simulink model "tcptank"  (R2024a)
settings: Solver=ode45  StartTime=0.0  StopTime=200.0  RelTol=1e-3  EnableMultiTasking=on
undefined symbols (not defined in the file): DiscIntNeverNeededParam, Ts
libraries: instrumentlib x4, simulink x3, rllib x1
settings Model: Creator=The MathWorks, Inc.  LastModifiedBy=Administrator
settings SolverCC: AlgebraicLoopSolver=TrustRegion
settings DataIOCC: LimitDataPoints=on  SaveFormat=Array  ReturnWorkspaceOutputs=off  SignalLoggingName=logsOut
settings OptimizationCC: ExpressionDepthLimit=2147483647  InitFltsAndDblsToZero=on  LifeSpan=inf
settings DebuggingCC: SaveWithParameterizedLinksMsg=none  UnderspecifiedInitializationDetection=Classic  MergeDetectMultiDrivingBlocksExec=none  SignalResolutionControl=TryResolveAllWithWarning  MultiTaskDSMMsg=warning  FcnCallInpInsideContextMsg=warning  UnconnectedInputMsg=warning  UnconnectedOutputMsg=warning  UnconnectedLineMsg=warning  AllowSymbolicDim=off  StateNameClashWarn=warning  SFUnexpectedBacktrackingDiag=warning  SFNoUnconditionalDefaultTransitionDiag=warning  SFExecutionAtInitializationDiag=none  ArithmeticOperatorsInVariantConditions=warning
settings HardwareCC: ProdBitPerPointer=32  ProdBitPerSizeT=32  ProdBitPerPtrDiffT=32  ProdLargestAtomicFloat=None  ProdIntDivRoundTo=Undefined  ProdEndianess=Unspecified  ProdWordSize=32  ProdHWDeviceType=Specified
settings ModelReferenceCC: EnableRefExpFcnMdlSchedulingChecks=on  PropagateSignalLabelsOutOfModel=off
settings SFSimCC: SimUseLocalCustomCode=off
settings RTWCC: RTWUseLocalCustomCode=off  GPUComputeCapability=3.5
settings CodeAppCC: StateflowObjectComments=on
settings GRTTargetCC: TargetFcnLib=ansi_tfl_tmw.mat  TargetLangStandard=C89/C90 (ANSI)  CombineOutputUpdateFcns=off  GRTInterface=on
settings ConfigComp: CovMetricSettings=dw  CovSaveCumulativeToWorkspaceVar=on  CovSaveSingleToWorkspaceVar=on  CovExternalEMLEnable=off

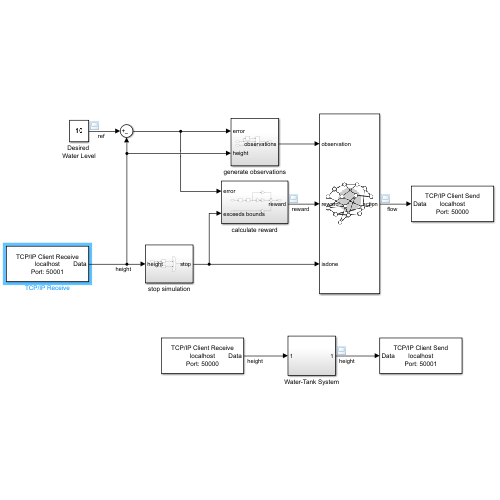
[thumbnail: Simulink's stored preview of the top-level diagram]
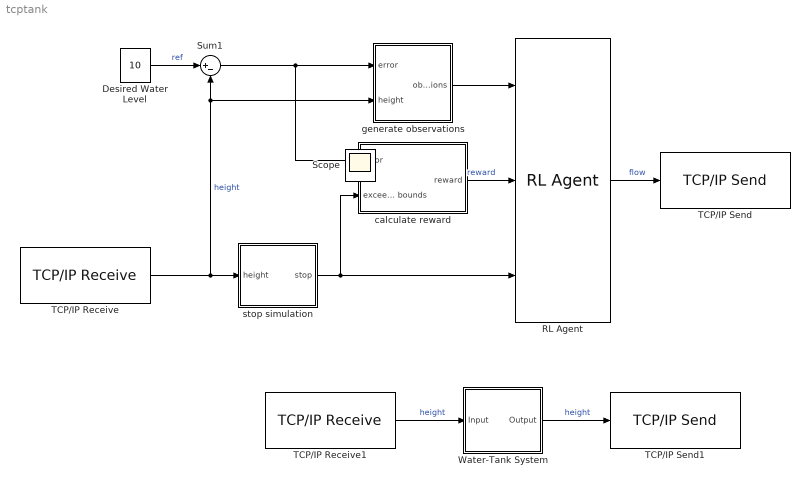
== system tcptank ==
  Desired Water Level : Constant  Value=10
  RL Agent : rllib/RL Agent  Agent=agent  ExternalActionAsInput=off  ProvideLastAction=off  ProvideCumRwd=off  TreatAsDirectFeedthrough=on  UseStrictObservationDataTypes=off
  Sum1 : Sum  Inputs=|+-  SaturateOnIntegerOverflow=on
  TCP/IP Receive : instrumentlib/TCP//IP Receive  Host=localhost  Port=50001  DataSize=[ 1, 1 ]  DataType=double  ASCIIFormatting=%f  Terminator=LF  CustomTerminator=10  ByteOrder=big-endian  EnableBlockingMode=on  Timeout=10  SampleTime=0.01  SimulateUsing=Interpreted execution
  TCP/IP Receive1 : instrumentlib/TCP//IP Receive  Host=localhost  Port=50000  DataSize=[ 1, 1 ]  DataType=double  ASCIIFormatting=%f  Terminator=LF  CustomTerminator=10  ByteOrder=big-endian  EnableBlockingMode=on  Timeout=10  SampleTime=0.01  SimulateUsing=Interpreted execution
  TCP/IP Send : instrumentlib/TCP//IP Send  Host=localhost  Port=50000  ByteOrder=big-endian  EnableBlockingMode=on  Timeout=10  TransferDelay=on  SimulateUsing=Interpreted execution
  TCP/IP Send1 : instrumentlib/TCP//IP Send  Host=localhost  Port=50001  ByteOrder=big-endian  EnableBlockingMode=on  Timeout=10  TransferDelay=on  SimulateUsing=Interpreted execution
  Water-Tank System : Subsystem
  calculate reward : Subsystem
  generate observations : Subsystem
  stop simulation : Subsystem
  Scope : Scope
  wires:
  Desired Water Level/1 -> Sum1/1  "ref"
  Sum1/1 -> calculate reward/1(error), generate observations/1(error)
  TCP/IP Receive/1 -> stop simulation/1(height), generate observations/2(height), Sum1/2  "height"
  RL Agent/1 -> TCP/IP Send/1  "flow"
  stop simulation/1(stop) -> RL Agent/3, calculate reward/2(exceeds bounds)
  calculate reward/1(reward) -> RL Agent/2  "reward"
  generate observations/1(observations) -> RL Agent/1
  TCP/IP Receive1/1 -> Water-Tank System/1(Input)  "height"
  Water-Tank System/1(Output) -> TCP/IP Send1/1  "height"

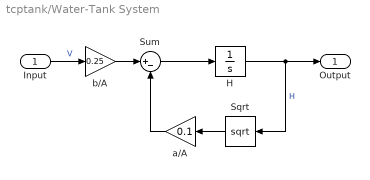
== system tcptank/Water-Tank System ==
  Input : Inport
  H : Integrator  InitialCondition=3  LimitOutput=on  LowerSaturationLimit=0
  Sqrt : Sqrt  OutputSignalType=real
  Sum : Sum  Inputs=|+-  SaturateOnIntegerOverflow=on
  a/A : Gain  Gain=0.1  SaturateOnIntegerOverflow=on  OutDataTypeStr=Inherit: Same as input  ParamDataTypeStr=Inherit: Same as input
  b/A : Gain  Gain=0.25  SaturateOnIntegerOverflow=on  OutDataTypeStr=Inherit: Same as input  ParamDataTypeStr=Inherit: Same as input
  Output : Outport  VectorParamsAs1DForOutWhenUnconnected=off
  wires:
  b/A/1 -> Sum/1
  Sum/1 -> H/1
  H/1 -> Sqrt/1, Output/1  "H"
  Sqrt/1 -> a/A/1
  a/A/1 -> Sum/2
  Input/1 -> b/A/1  "V"

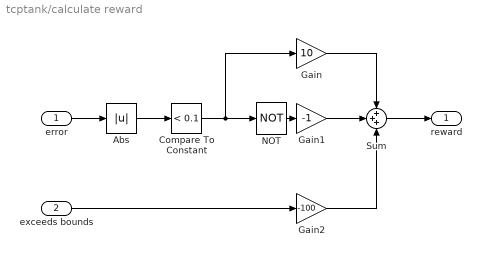
== system tcptank/calculate reward ==
  error : Inport
  exceeds bounds : Inport  Port=2
  Abs : Abs  SaturateOnIntegerOverflow=off
  Compare To Constant : simulink/Logic and Bit Operations/Compare To Constant  relop=<  const=0.1  OutDataTypeStr=boolean
  Gain : Gain  Gain=10
  Gain1 : Gain  Gain=-1
  Gain2 : Gain  Gain=-100
  NOT : Logic  Operator=NOT  IconShape=distinctive  AllPortsSameDT=off  OutDataTypeStr=boolean
  Sum : Sum  Inputs=+++  OutDataTypeStr=double
  reward : Outport  VectorParamsAs1DForOutWhenUnconnected=off
  wires:
  Abs/1 -> Compare To Constant/1
  Gain2/1 -> Sum/3
  Gain/1 -> Sum/1
  Compare To Constant/1 -> NOT/1, Gain/1
  Gain1/1 -> Sum/2
  Sum/1 -> reward/1
  NOT/1 -> Gain1/1
  exceeds bounds/1 -> Gain2/1
  error/1 -> Abs/1

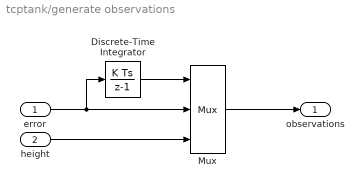
== system tcptank/generate observations ==
  error : Inport
  height : Inport  Port=2
  Discrete-Time Integrator : DiscreteIntegrator  SampleTime=Ts  ICPrevOutput=DiscIntNeverNeededParam  ICPrevScaledInput=DiscIntNeverNeededParam
  Mux : Mux  Inputs=3
  observations : Outport  VectorParamsAs1DForOutWhenUnconnected=off
  wires:
  height/1 -> Mux/3
  Discrete-Time Integrator/1 -> Mux/1
  error/1 -> Discrete-Time Integrator/1, Mux/2
  Mux/1 -> observations/1

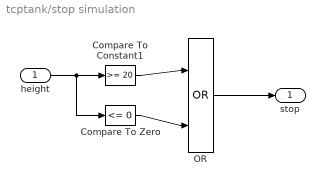
== system tcptank/stop simulation ==
  height : Inport
  Compare To Constant1 : simulink/Logic and Bit Operations/Compare To Constant  relop=>=  const=20  OutDataTypeStr=boolean
  Compare To Zero : simulink/Logic and Bit Operations/Compare To Zero  relop=<=  OutDataTypeStr=boolean
  OR : Logic  Operator=OR  IconShape=distinctive  AllPortsSameDT=off  OutDataTypeStr=boolean
  stop : Outport  VectorParamsAs1DForOutWhenUnconnected=off
  wires:
  height/1 -> Compare To Zero/1, Compare To Constant1/1
  Compare To Zero/1 -> OR/2
  Compare To Constant1/1 -> OR/1
  OR/1 -> stop/1
